simulink model "furuta_block_model"  (R2026b)
settings: Solver=FixedStepDiscrete  StopTime=5  FixedStep=controlPeriod
model workspace (MAT data in the model file):
  controlPeriod = 0.01
  initialState = [0; 0.174532925199; 0; 0]
  integrationStep = 0.002
  lqrGain = [-0.560244322113 -7.30813603654 -0.304541725168 -0.68699829167]
  maxTorque = 0.03
  plantCoefficients = [0.00019818 0.00016078 0.00016134 0.00013805 0.016934 0.0001 1e-05 0]
  scenarioStimulus = [0 0.0075 0.0175 0.0275 0.0375 0.0475 0.0575 0.0675 0.0775 0.0875 0.0975 0.1075 ... (2004 elements, 501x4)]
  usePolicyCallback = 0
values from neighbouring files (symbols this model uses):
  C = [B A*B A^2*B A^3*B]    [build_furuta_rmd.m]
  N = 20    [build_furuta_rl.m]    (also in design_classical.m)
  pidGains = getVariable(mw,'pidGains')    [check_furuta_lqr_capture.m]
  rmd = struct('model','RMD-X6-P20-60-E','voltage',48,'gearRatio',19.612,          'ratedTorque',20,'ratedCurrent',9.5,'ratedSpeedRPM',153,          'noLoadSpeedRPM',176,'Kt',2.1,'currentLSB',.01)    [build_furuta_rmd.m]
  s = load(matFile,'ds')    [analyze_pi_current_run.m]    (also in analyze_pi_speed_run.m; build_furuta_rl.m = sin(x(2));"; build_furuta_simulink.m = s(1); design_classical.m = furuta_scenarios)
  source = [step '/1']    [add_furuta_plant_blocks.m]    (also in build_furuta_pi.m = get_param(line,'SrcPortHandle'); build_furuta_pi_hardware.m = 'Drive interlocks/3'; compare_furuta_actuators.m = get_param([harness '/Requested torque'],'PortHandles'))
  Z = expm([A B; zeros(1,5)]*p.Ts)    [furuta_linearize.m]
undefined symbols (not defined in the file or in its folder): driveElectrical, lmpcF, lmpcH, poleGain, rlRewardLevel, rmdCommandDelaySamples, sgn, useRmd, X, Y
libraries: sm_lib x36, nesl_utility x8, fl_lib x7, rllib x2, mpclib x1, slpidlib x1, ee_lib x1
(part 3 of 4)

== system furuta_block_model/05 Furuta plant/RK4 Furuta plant ==
  state : Inport
  total torque : Inport  Port=2
  Substep 1 : Subsystem
  Substep 2 : Subsystem
  Substep 3 : Subsystem
  Substep 4 : Subsystem
  Substep 5 : Subsystem
  next state : Outport
  wires:
  state/1 -> Substep 1/1(x)
  total torque/1 -> Substep 4/2(tau), Substep 5/2(tau), Substep 3/2(tau), Substep 2/2(tau), Substep 1/2(tau)
  Substep 1/1(x next) -> Substep 2/1(x)
  Substep 2/1(x next) -> Substep 3/1(x)
  Substep 3/1(x next) -> Substep 4/1(x)
  Substep 4/1(x next) -> Substep 5/1(x)
  Substep 5/1(x next) -> next state/1

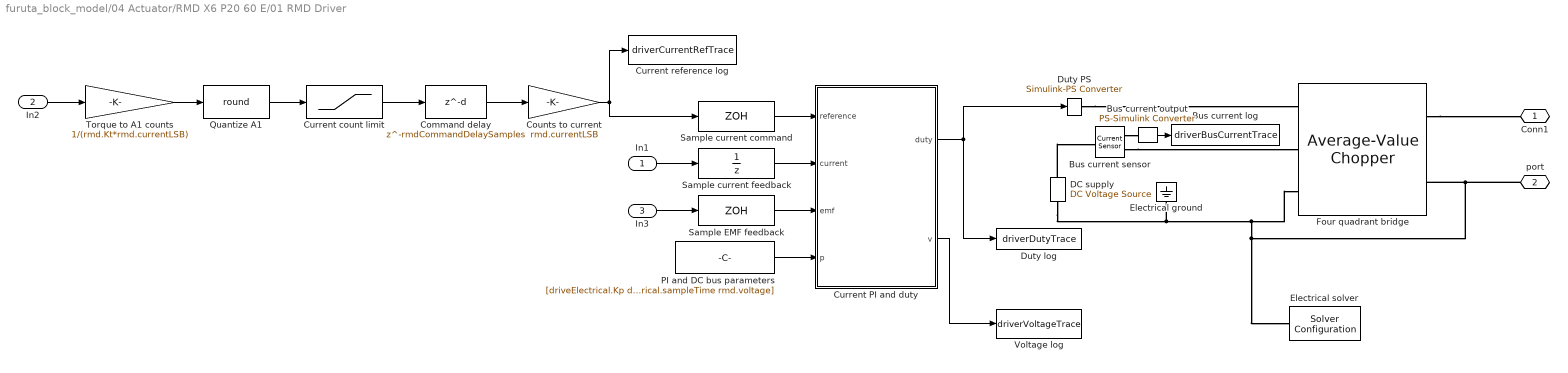
== system furuta_block_model/04 Actuator/RMD X6 P20 60 E/01 RMD Driver ==
  In1 : Inport
  In2 : Inport  Port=2
  In3 : Inport  Port=3
  Bus current log : ToWorkspace  VariableName=driverBusCurrentTrace  SaveFormat=Timeseries  SampleTime=-1
  Bus current output : nesl_utility/PS-Simulink Converter  PhysicalDomain=network_engine_domain  SubClassName=ps_output  LeftPortType=input  RightPortType=output  PseudoPeriodic=off  Frequencies=[]  VectorFormat=inherit  Unit=A  AffineConversion=off
  Bus current sensor : fl_lib/Electrical/Electrical Sensors/Current Sensor
  Command delay : Delay  DelayLength=rmdCommandDelaySamples  SampleTime=controlPeriod
  Counts to current : Gain  Gain=rmd.currentLSB
  Current PI and duty : MATLAB Function  TreatAsAtomicUnit=on
  Current count limit : Saturate  UpperLimit=floor(min([maxTorque/rmd.Kt rmd.ratedTorque/rmd.Kt rmd.ratedCurrent])/rmd.currentLSB)  LowerLimit=-(floor(min([maxTorque/rmd.Kt rmd.ratedTorque/rmd.Kt rmd.ratedCurrent])/rmd.currentLSB))
  Current reference log : ToWorkspace  VariableName=driverCurrentRefTrace  SaveFormat=Timeseries  SampleTime=-1
  DC supply : fl_lib/Electrical/Electrical Sources/DC Voltage Source  v0=rmd.voltage V
  Duty PS : nesl_utility/Simulink-PS Converter  PhysicalDomain=network_engine_domain  SubClassName=ps_input  LeftPortType=input  RightPortType=output  PseudoPeriodic=off  Frequencies=[]  NoiseDistribution=none  NoiseParameters=[]  Unit=1  AffineConversion=off  FilteringAndDerivatives=zero  SimscapeFilterOrder=1  InputFilterTimeConstant=0.001  UdotUserProvided=0
  Duty log : ToWorkspace  VariableName=driverDutyTrace  SaveFormat=Timeseries  SampleTime=-1
  Electrical ground : fl_lib/Electrical/Electrical Elements/Electrical Reference
  Electrical solver : nesl_utility/Solver Configuration  PhysicalDomain=network_engine_domain  SubClassName=solver  LeftPortType=input  RightPortType=generic  Tones=[]  Harmonics=[]  SimulateNoise=off  Profile=off  UseLocalSampling=off  EnableSwitchedLinearOptims=on  FrequencyDomain=off  UseCCode=off  RelTol=0.001  AbsTol=0.001  MinStep=1e-09  ToWorkspace=off  RevertToSquareIcSolve=off  NumHomotopyIterations=100  PhasorMode=off  PhasorModeNumHarmonics=1  ConsistencySolver=NEWTON_XTOL_AFTER_FTOL  CanonicalOrdering=CANONICAL  OptimizeIntermediates=OPTIMIZED  MulticoreSolverChoice=BACKWARD_EULER  IndexReductionMethod=DerivativeReplacement  DoDC=off  ResidualTolerance=1e-09  ConsistencyTolSource=GLOBAL  ConsistencyAbsTol=0.001  ConsistencyRelTol=0.001  ConsistencyTolFactor=0.001  UseLocalSolver=off  LocalSolverChoice=NE_BACKWARD_EULER_ADVANCER  ResolveIndetEquations=on  FunctionEvalNumThread=1  LocalSolverSampleTime=0.001  DoFixedCost=off  MaxNonlinIter=3  MaxModeIter=2  ComputeImpulses=off  ImpulseIterations=2  LinearAlgebra=auto  LinearAlgebraNumThread=0  EquationFormulation=NE_TIME_EF  DelaysMemoryBudget=1024  AutomaticFiltering=on  FilteringTimeConstant=0.001  PartitionStorageMethod=AS_NEEDED  PartitionMemoryBudget=1024  PartitionMethod=BALANCED  MultibodyUseLocalSolver=off  MultibodyLocalSolverChoice=ODE1  MultibodyLocalSolverSampleTime=0.001
  Four quadrant bridge : ee_lib/Semiconductors & Converters/Converters/Average-Value Chopper  chopper_type=ee.enum.converters.averageChopperType.classE  efficiency_option=ee.enum.converters.efficiencyOption.constant  efficiency_fixed=100  i_vec=[0, 2, 5] A  efficiency_vec=[90, 95, 98]
  PI and DC bus parameters : Constant  Value=[driveElectrical.Kp driveElectrical.Ki driveElectrical.sampleTime rmd.voltage]
  Quantize A1 : Rounding  Operator=round
  Sample EMF feedback : ZeroOrderHold  SampleTime=driveElectrical.sampleTime
  Sample current command : ZeroOrderHold  SampleTime=driveElectrical.sampleTime
  Sample current feedback : UnitDelay  SampleTime=driveElectrical.sampleTime
  Torque to A1 counts : Gain  Gain=1/(rmd.Kt*rmd.currentLSB)
  Voltage log : ToWorkspace  VariableName=driverVoltageTrace  SaveFormat=Timeseries  SampleTime=-1
  Conn1 : PMIOPort  Side=Right
  port : PMIOPort  Port=2  Side=Left
  wires:
  Torque to A1 counts/1 -> Quantize A1/1
  Command delay/1 -> Counts to current/1
  Bus current output/1 -> Bus current log/1
  Sample current command/1 -> Current PI and duty/1(reference)
  Counts to current/1 -> Current reference log/1, Sample current command/1
  Current count limit/1 -> Command delay/1
  Quantize A1/1 -> Current count limit/1
  Current PI and duty/1(duty) -> Duty PS/1, Duty log/1
  Sample current feedback/1 -> Current PI and duty/2(current)
  In3/1 -> Sample EMF feedback/1
  Current PI and duty/2(v) -> Voltage log/1
  Sample EMF feedback/1 -> Current PI and duty/3(emf)
  PI and DC bus parameters/1 -> Current PI and duty/4(p)
  In1/1 -> Sample current feedback/1
  In2/1 -> Torque to A1 counts/1
  connections:
  Bus current sensor/RConn1 -- Bus current output/LConn1
  port/RConn1 -- Four quadrant bridge/RConn2 -- Electrical solver/RConn1 -- Four quadrant bridge/LConn3 -- DC supply/RConn1 -- Electrical ground/LConn1
  Duty PS/RConn1 -- Four quadrant bridge/LConn1
  DC supply/LConn1 -- Bus current sensor/LConn1
  Bus current sensor/RConn2 -- Four quadrant bridge/LConn2
  Four quadrant bridge/RConn1 -- Conn1/RConn1

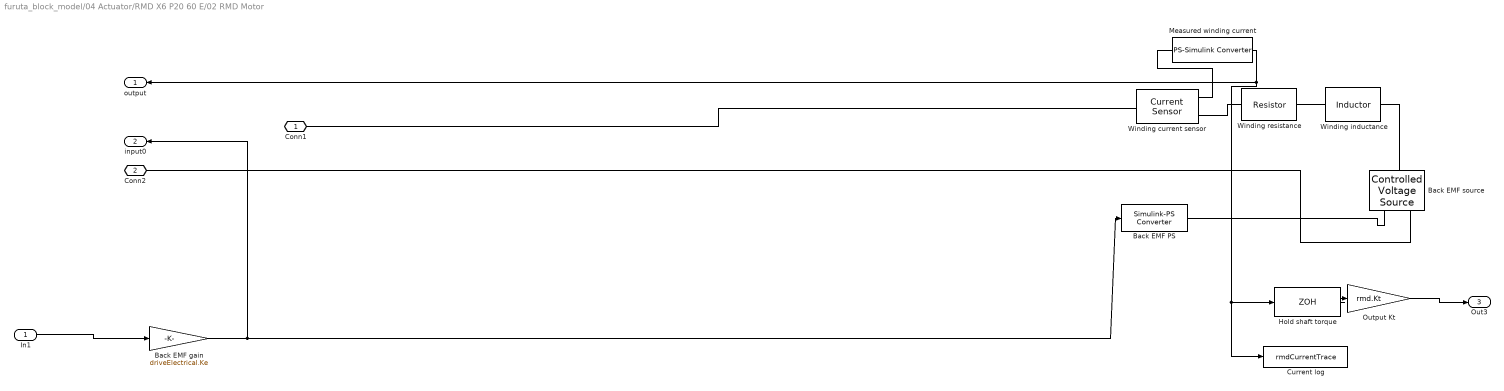
== system furuta_block_model/04 Actuator/RMD X6 P20 60 E/02 RMD Motor ==
  In1 : Inport
  Back EMF PS : nesl_utility/Simulink-PS Converter  PhysicalDomain=network_engine_domain  SubClassName=ps_input  LeftPortType=input  RightPortType=output  PseudoPeriodic=off  Frequencies=[]  NoiseDistribution=none  NoiseParameters=[]  Unit=V  AffineConversion=off  FilteringAndDerivatives=zero  SimscapeFilterOrder=1  InputFilterTimeConstant=0.001  UdotUserProvided=0
  Back EMF gain : Gain  Gain=driveElectrical.Ke
  Back EMF source : fl_lib/Electrical/Electrical Sources/Controlled Voltage Source
  Current log : ToWorkspace  VariableName=rmdCurrentTrace  SampleTime=-1
  Hold shaft torque : ZeroOrderHold  SampleTime=controlPeriod
  Measured winding current : nesl_utility/PS-Simulink Converter  PhysicalDomain=network_engine_domain  SubClassName=ps_output  LeftPortType=input  RightPortType=output  PseudoPeriodic=off  Frequencies=[]  VectorFormat=inherit  Unit=A  AffineConversion=off
  Output Kt : Gain  Gain=rmd.Kt
  Winding current sensor : fl_lib/Electrical/Electrical Sensors/Current Sensor
  Winding inductance : fl_lib/Electrical/Electrical Elements/Inductor  l=driveElectrical.L H  r=0 Ohm  g=0 1/Ohm  i_specify=off  i_priority=None  i=0 A  i_nominal_specify=off  i_nominal_value=1  i_nominal_unit=A  v_specify=off  v_priority=None  v=0 V  v_nominal_specify=off  v_nominal_value=1  v_nominal_unit=V  i_L_specify=off  i_L_priority=High  i_L=0 A  i_L_nominal_specify=off  i_L_nominal_value=1  i_L_nominal_unit=A
  Winding resistance : fl_lib/Electrical/Electrical Elements/Resistor  R=driveElectrical.R Ohm  i_specify=off  i_priority=None  i=0 A  i_nominal_specify=off  i_nominal_value=1  i_nominal_unit=A  v_specify=off  v_priority=None  v=0 V  v_nominal_specify=off  v_nominal_value=1  v_nominal_unit=V
  Conn1 : PMIOPort  Side=Left
  Conn2 : PMIOPort  Port=2  Side=Right
  output : Outport
  input0 : Outport  Port=2
  Out3 : Outport  Port=3
  wires:
  Measured winding current/1 -> output/1, Hold shaft torque/1, Current log/1
  Output Kt/1 -> Out3/1
  Hold shaft torque/1 -> Output Kt/1
  Back EMF gain/1 -> Back EMF PS/1, input0/1
  In1/1 -> Back EMF gain/1
  connections:
  Back EMF PS/RConn1 -- Back EMF source/RConn1
  Winding current sensor/RConn1 -- Measured winding current/LConn1
  Winding resistance/RConn1 -- Winding inductance/LConn1
  Winding inductance/RConn1 -- Back EMF source/LConn1
  Winding current sensor/RConn2 -- Winding resistance/LConn1
  Conn1/RConn1 -- Winding current sensor/LConn1
  Back EMF source/RConn2 -- Conn2/RConn1

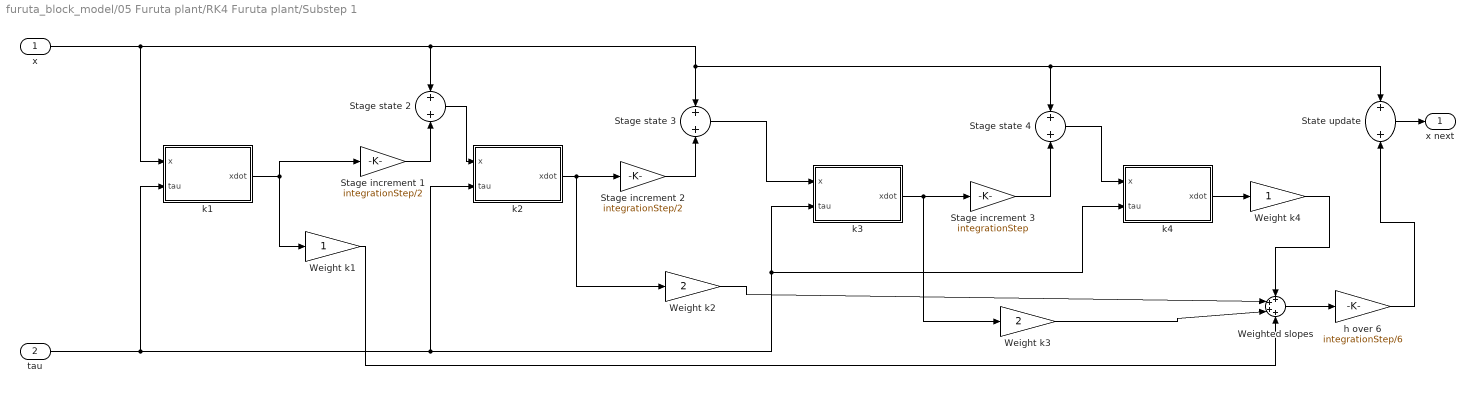
== system furuta_block_model/05 Furuta plant/RK4 Furuta plant/Substep 1 ==
  x : Inport
  tau : Inport  Port=2
  Stage increment 1 : Gain  Gain=integrationStep/2
  Stage increment 2 : Gain  Gain=integrationStep/2
  Stage increment 3 : Gain  Gain=integrationStep
  Stage state 2 : Sum
  Stage state 3 : Sum
  Stage state 4 : Sum
  State update : Sum
  Weight k1 : Gain
  Weight k2 : Gain  Gain=2
  Weight k3 : Gain  Gain=2
  Weight k4 : Gain
  Weighted slopes : Sum  Inputs=++++
  h over 6 : Gain  Gain=integrationStep/6
  k1 : Subsystem
  k2 : Subsystem
  k3 : Subsystem
  k4 : Subsystem
  x next : Outport
  wires:
  x/1 -> Stage state 3/1, Stage state 4/1, State update/1, Stage state 2/1, k1/1(x)
  tau/1 -> k4/2(tau), k3/2(tau), k2/2(tau), k1/2(tau)
  k1/1(xdot) -> Stage increment 1/1, Weight k1/1
  Stage increment 1/1 -> Stage state 2/2
  Stage state 2/1 -> k2/1(x)
  k2/1(xdot) -> Stage increment 2/1, Weight k2/1
  Stage increment 2/1 -> Stage state 3/2
  Stage state 3/1 -> k3/1(x)
  k3/1(xdot) -> Weight k3/1, Stage increment 3/1
  Stage increment 3/1 -> Stage state 4/2
  Stage state 4/1 -> k4/1(x)
  k4/1(xdot) -> Weight k4/1
  Weight k1/1 -> Weighted slopes/4
  Weight k2/1 -> Weighted slopes/2
  Weight k3/1 -> Weighted slopes/3
  Weight k4/1 -> Weighted slopes/1
  Weighted slopes/1 -> h over 6/1
  h over 6/1 -> State update/2
  State update/1 -> x next/1

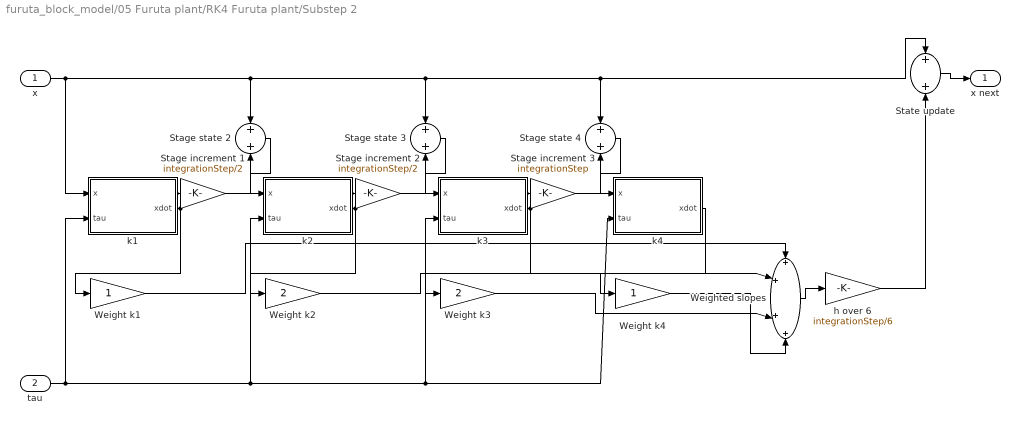
== system furuta_block_model/05 Furuta plant/RK4 Furuta plant/Substep 2 ==
  x : Inport
  tau : Inport  Port=2
  Stage increment 1 : Gain  Gain=integrationStep/2
  Stage increment 2 : Gain  Gain=integrationStep/2
  Stage increment 3 : Gain  Gain=integrationStep
  Stage state 2 : Sum
  Stage state 3 : Sum
  Stage state 4 : Sum
  State update : Sum
  Weight k1 : Gain
  Weight k2 : Gain  Gain=2
  Weight k3 : Gain  Gain=2
  Weight k4 : Gain
  Weighted slopes : Sum  Inputs=++++
  h over 6 : Gain  Gain=integrationStep/6
  k1 : Subsystem
  k2 : Subsystem
  k3 : Subsystem
  k4 : Subsystem
  x next : Outport
  wires:
  State update/1 -> x next/1
  h over 6/1 -> State update/2
  Weighted slopes/1 -> h over 6/1
  Weight k4/1 -> Weighted slopes/4
  Weight k3/1 -> Weighted slopes/3
  Weight k2/1 -> Weighted slopes/2
  Weight k1/1 -> Weighted slopes/1
  k4/1(xdot) -> Weight k4/1
  Stage state 4/1 -> k4/1(x)
  Stage increment 3/1 -> Stage state 4/2
  k3/1(xdot) -> Weight k3/1, Stage increment 3/1
  Stage state 3/1 -> k3/1(x)
  Stage increment 2/1 -> Stage state 3/2
  k2/1(xdot) -> Weight k2/1, Stage increment 2/1
  Stage state 2/1 -> k2/1(x)
  Stage increment 1/1 -> Stage state 2/2
  k1/1(xdot) -> Weight k1/1, Stage increment 1/1
  tau/1 -> k4/2(tau), k3/2(tau), k2/2(tau), k1/2(tau)
  x/1 -> State update/1, Stage state 4/1, Stage state 3/1, Stage state 2/1, k1/1(x)

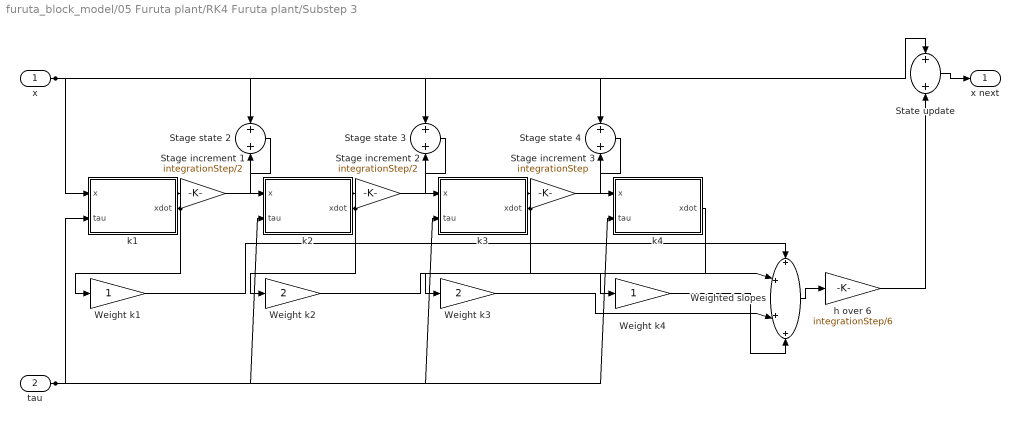
== system furuta_block_model/05 Furuta plant/RK4 Furuta plant/Substep 3 ==
  x : Inport
  tau : Inport  Port=2
  Stage increment 1 : Gain  Gain=integrationStep/2
  Stage increment 2 : Gain  Gain=integrationStep/2
  Stage increment 3 : Gain  Gain=integrationStep
  Stage state 2 : Sum
  Stage state 3 : Sum
  Stage state 4 : Sum
  State update : Sum
  Weight k1 : Gain
  Weight k2 : Gain  Gain=2
  Weight k3 : Gain  Gain=2
  Weight k4 : Gain
  Weighted slopes : Sum  Inputs=++++
  h over 6 : Gain  Gain=integrationStep/6
  k1 : Subsystem
  k2 : Subsystem
  k3 : Subsystem
  k4 : Subsystem
  x next : Outport
  wires:
  State update/1 -> x next/1
  h over 6/1 -> State update/2
  Weighted slopes/1 -> h over 6/1
  Weight k4/1 -> Weighted slopes/4
  Weight k3/1 -> Weighted slopes/3
  Weight k2/1 -> Weighted slopes/2
  Weight k1/1 -> Weighted slopes/1
  k4/1(xdot) -> Weight k4/1
  Stage state 4/1 -> k4/1(x)
  Stage increment 3/1 -> Stage state 4/2
  k3/1(xdot) -> Weight k3/1, Stage increment 3/1
  Stage state 3/1 -> k3/1(x)
  Stage increment 2/1 -> Stage state 3/2
  k2/1(xdot) -> Weight k2/1, Stage increment 2/1
  Stage state 2/1 -> k2/1(x)
  Stage increment 1/1 -> Stage state 2/2
  k1/1(xdot) -> Weight k1/1, Stage increment 1/1
  tau/1 -> k4/2(tau), k3/2(tau), k2/2(tau), k1/2(tau)
  x/1 -> State update/1, Stage state 4/1, Stage state 3/1, Stage state 2/1, k1/1(x)

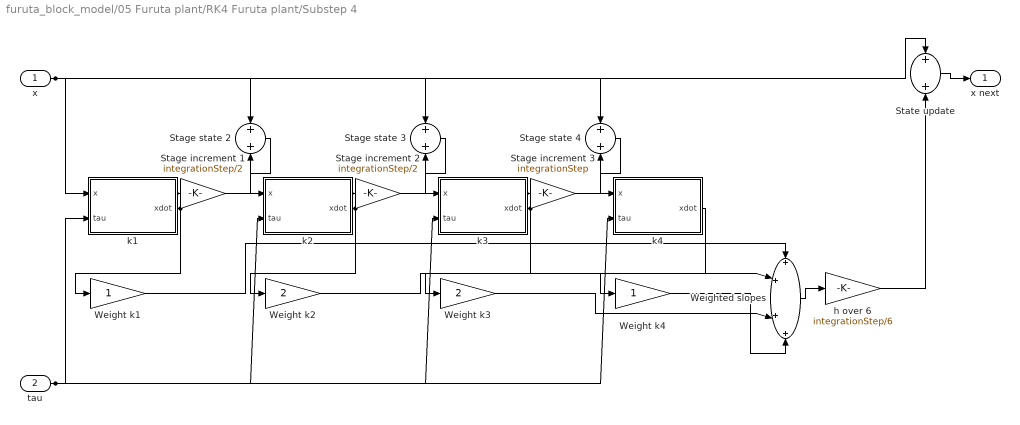
== system furuta_block_model/05 Furuta plant/RK4 Furuta plant/Substep 4 ==
  x : Inport
  tau : Inport  Port=2
  Stage increment 1 : Gain  Gain=integrationStep/2
  Stage increment 2 : Gain  Gain=integrationStep/2
  Stage increment 3 : Gain  Gain=integrationStep
  Stage state 2 : Sum
  Stage state 3 : Sum
  Stage state 4 : Sum
  State update : Sum
  Weight k1 : Gain
  Weight k2 : Gain  Gain=2
  Weight k3 : Gain  Gain=2
  Weight k4 : Gain
  Weighted slopes : Sum  Inputs=++++
  h over 6 : Gain  Gain=integrationStep/6
  k1 : Subsystem
  k2 : Subsystem
  k3 : Subsystem
  k4 : Subsystem
  x next : Outport
  wires:
  State update/1 -> x next/1
  h over 6/1 -> State update/2
  Weighted slopes/1 -> h over 6/1
  Weight k4/1 -> Weighted slopes/4
  Weight k3/1 -> Weighted slopes/3
  Weight k2/1 -> Weighted slopes/2
  Weight k1/1 -> Weighted slopes/1
  k4/1(xdot) -> Weight k4/1
  Stage state 4/1 -> k4/1(x)
  Stage increment 3/1 -> Stage state 4/2
  k3/1(xdot) -> Weight k3/1, Stage increment 3/1
  Stage state 3/1 -> k3/1(x)
  Stage increment 2/1 -> Stage state 3/2
  k2/1(xdot) -> Weight k2/1, Stage increment 2/1
  Stage state 2/1 -> k2/1(x)
  Stage increment 1/1 -> Stage state 2/2
  k1/1(xdot) -> Weight k1/1, Stage increment 1/1
  tau/1 -> k4/2(tau), k3/2(tau), k2/2(tau), k1/2(tau)
  x/1 -> State update/1, Stage state 4/1, Stage state 3/1, Stage state 2/1, k1/1(x)

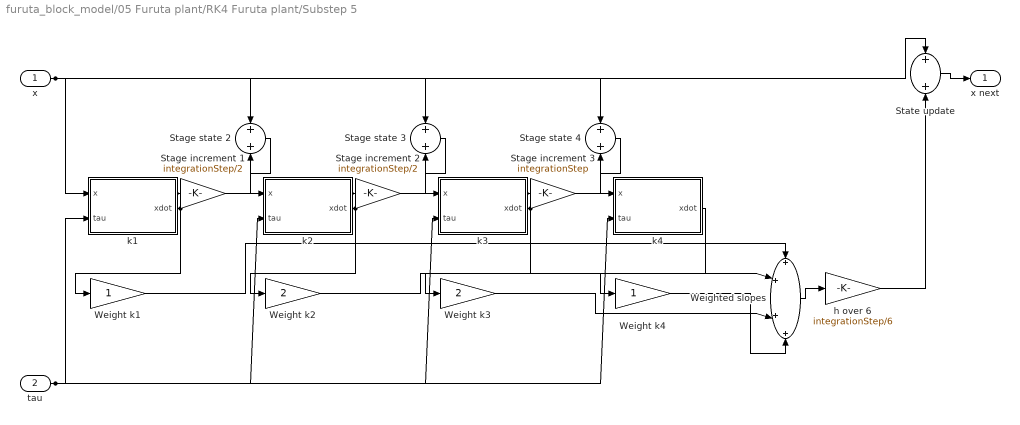
== system furuta_block_model/05 Furuta plant/RK4 Furuta plant/Substep 5 ==
  x : Inport
  tau : Inport  Port=2
  Stage increment 1 : Gain  Gain=integrationStep/2
  Stage increment 2 : Gain  Gain=integrationStep/2
  Stage increment 3 : Gain  Gain=integrationStep
  Stage state 2 : Sum
  Stage state 3 : Sum
  Stage state 4 : Sum
  State update : Sum
  Weight k1 : Gain
  Weight k2 : Gain  Gain=2
  Weight k3 : Gain  Gain=2
  Weight k4 : Gain
  Weighted slopes : Sum  Inputs=++++
  h over 6 : Gain  Gain=integrationStep/6
  k1 : Subsystem
  k2 : Subsystem
  k3 : Subsystem
  k4 : Subsystem
  x next : Outport
  wires:
  State update/1 -> x next/1
  h over 6/1 -> State update/2
  Weighted slopes/1 -> h over 6/1
  Weight k4/1 -> Weighted slopes/4
  Weight k3/1 -> Weighted slopes/3
  Weight k2/1 -> Weighted slopes/2
  Weight k1/1 -> Weighted slopes/1
  k4/1(xdot) -> Weight k4/1
  Stage state 4/1 -> k4/1(x)
  Stage increment 3/1 -> Stage state 4/2
  k3/1(xdot) -> Weight k3/1, Stage increment 3/1
  Stage state 3/1 -> k3/1(x)
  Stage increment 2/1 -> Stage state 3/2
  k2/1(xdot) -> Weight k2/1, Stage increment 2/1
  Stage state 2/1 -> k2/1(x)
  Stage increment 1/1 -> Stage state 2/2
  k1/1(xdot) -> Weight k1/1, Stage increment 1/1
  tau/1 -> k4/2(tau), k3/2(tau), k2/2(tau), k1/2(tau)
  x/1 -> State update/1, Stage state 4/1, Stage state 3/1, Stage state 2/1, k1/1(x)

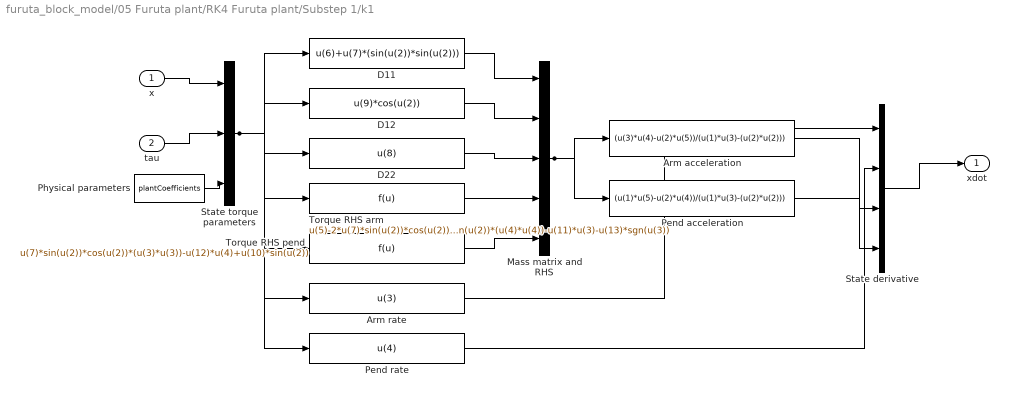
== system furuta_block_model/05 Furuta plant/RK4 Furuta plant/Substep 1/k1 ==
  x : Inport
  tau : Inport  Port=2
  Arm acceleration : Fcn  Expr=(u(3)*u(4)-u(2)*u(5))/(u(1)*u(3)-(u(2)*u(2)))
  Arm rate : Fcn  Expr=u(3)
  D11 : Fcn  Expr=u(6)+u(7)*(sin(u(2))*sin(u(2)))
  D12 : Fcn  Expr=u(9)*cos(u(2))
  D22 : Fcn  Expr=u(8)
  Mass matrix and RHS : Mux  Inputs=5
  Pend acceleration : Fcn  Expr=(u(1)*u(5)-u(2)*u(4))/(u(1)*u(3)-(u(2)*u(2)))
  Pend rate : Fcn  Expr=u(4)
  Physical parameters : Constant  Value=plantCoefficients
  State derivative : Mux
  State torque parameters : Mux  Inputs=3
  Torque RHS arm : Fcn  Expr=u(5)-2*u(7)*sin(u(2))*cos(u(2))*u(3)*u(4)+u(9)*sin(u(2))*(u(4)*u(4))-u(11)*u(3)-u(13)*sgn(u(3))
  Torque RHS pend : Fcn  Expr=u(7)*sin(u(2))*cos(u(2))*(u(3)*u(3))-u(12)*u(4)+u(10)*sin(u(2))
  xdot : Outport
  wires:
  x/1 -> State torque parameters/1
  tau/1 -> State torque parameters/2
  Physical parameters/1 -> State torque parameters/3
  State torque parameters/1 -> D11/1, D12/1, D22/1, Torque RHS arm/1, Torque RHS pend/1, Arm rate/1, Pend rate/1
  D11/1 -> Mass matrix and RHS/1
  D12/1 -> Mass matrix and RHS/2
  D22/1 -> Mass matrix and RHS/3
  Torque RHS arm/1 -> Mass matrix and RHS/4
  Torque RHS pend/1 -> Mass matrix and RHS/5
  Arm rate/1 -> State derivative/1
  Pend rate/1 -> State derivative/2
  Mass matrix and RHS/1 -> Arm acceleration/1, Pend acceleration/1
  Arm acceleration/1 -> State derivative/3
  Pend acceleration/1 -> State derivative/4
  State derivative/1 -> xdot/1

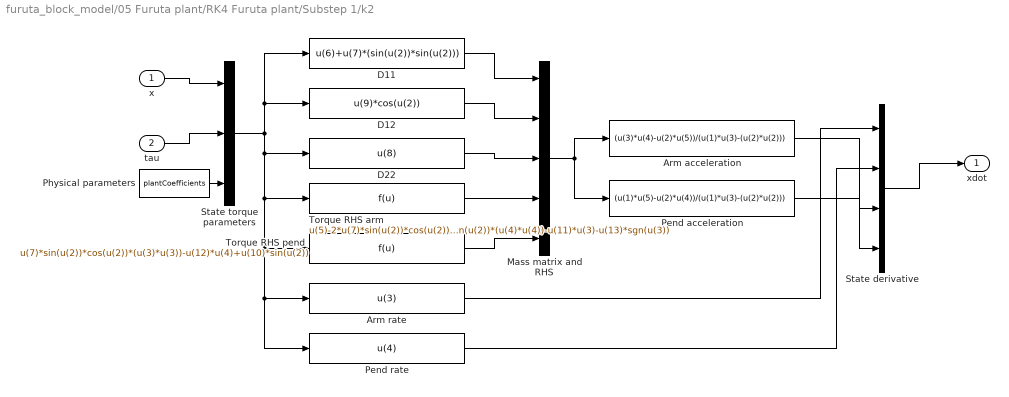
== system furuta_block_model/05 Furuta plant/RK4 Furuta plant/Substep 1/k2 ==
  x : Inport
  tau : Inport  Port=2
  Arm acceleration : Fcn  Expr=(u(3)*u(4)-u(2)*u(5))/(u(1)*u(3)-(u(2)*u(2)))
  Arm rate : Fcn  Expr=u(3)
  D11 : Fcn  Expr=u(6)+u(7)*(sin(u(2))*sin(u(2)))
  D12 : Fcn  Expr=u(9)*cos(u(2))
  D22 : Fcn  Expr=u(8)
  Mass matrix and RHS : Mux  Inputs=5
  Pend acceleration : Fcn  Expr=(u(1)*u(5)-u(2)*u(4))/(u(1)*u(3)-(u(2)*u(2)))
  Pend rate : Fcn  Expr=u(4)
  Physical parameters : Constant  Value=plantCoefficients
  State derivative : Mux
  State torque parameters : Mux  Inputs=3
  Torque RHS arm : Fcn  Expr=u(5)-2*u(7)*sin(u(2))*cos(u(2))*u(3)*u(4)+u(9)*sin(u(2))*(u(4)*u(4))-u(11)*u(3)-u(13)*sgn(u(3))
  Torque RHS pend : Fcn  Expr=u(7)*sin(u(2))*cos(u(2))*(u(3)*u(3))-u(12)*u(4)+u(10)*sin(u(2))
  xdot : Outport
  wires:
  State derivative/1 -> xdot/1
  Pend acceleration/1 -> State derivative/4
  Arm acceleration/1 -> State derivative/3
  Mass matrix and RHS/1 -> Pend acceleration/1, Arm acceleration/1
  Pend rate/1 -> State derivative/2
  Arm rate/1 -> State derivative/1
  Torque RHS pend/1 -> Mass matrix and RHS/5
  Torque RHS arm/1 -> Mass matrix and RHS/4
  D22/1 -> Mass matrix and RHS/3
  D12/1 -> Mass matrix and RHS/2
  D11/1 -> Mass matrix and RHS/1
  State torque parameters/1 -> Pend rate/1, Arm rate/1, Torque RHS pend/1, Torque RHS arm/1, D22/1, D12/1, D11/1
  Physical parameters/1 -> State torque parameters/3
  tau/1 -> State torque parameters/2
  x/1 -> State torque parameters/1

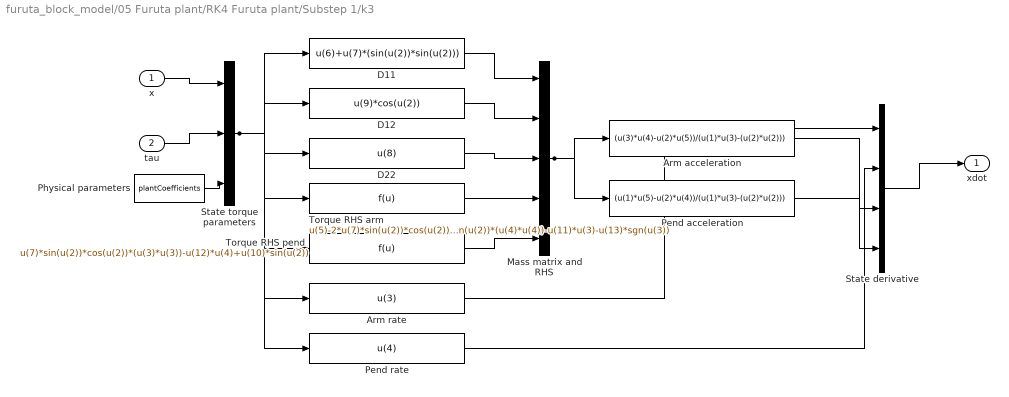
== system furuta_block_model/05 Furuta plant/RK4 Furuta plant/Substep 1/k3 ==
  x : Inport
  tau : Inport  Port=2
  Arm acceleration : Fcn  Expr=(u(3)*u(4)-u(2)*u(5))/(u(1)*u(3)-(u(2)*u(2)))
  Arm rate : Fcn  Expr=u(3)
  D11 : Fcn  Expr=u(6)+u(7)*(sin(u(2))*sin(u(2)))
  D12 : Fcn  Expr=u(9)*cos(u(2))
  D22 : Fcn  Expr=u(8)
  Mass matrix and RHS : Mux  Inputs=5
  Pend acceleration : Fcn  Expr=(u(1)*u(5)-u(2)*u(4))/(u(1)*u(3)-(u(2)*u(2)))
  Pend rate : Fcn  Expr=u(4)
  Physical parameters : Constant  Value=plantCoefficients
  State derivative : Mux
  State torque parameters : Mux  Inputs=3
  Torque RHS arm : Fcn  Expr=u(5)-2*u(7)*sin(u(2))*cos(u(2))*u(3)*u(4)+u(9)*sin(u(2))*(u(4)*u(4))-u(11)*u(3)-u(13)*sgn(u(3))
  Torque RHS pend : Fcn  Expr=u(7)*sin(u(2))*cos(u(2))*(u(3)*u(3))-u(12)*u(4)+u(10)*sin(u(2))
  xdot : Outport
  wires:
  State derivative/1 -> xdot/1
  Pend acceleration/1 -> State derivative/4
  Arm acceleration/1 -> State derivative/3
  Mass matrix and RHS/1 -> Pend acceleration/1, Arm acceleration/1
  Pend rate/1 -> State derivative/2
  Arm rate/1 -> State derivative/1
  Torque RHS pend/1 -> Mass matrix and RHS/5
  Torque RHS arm/1 -> Mass matrix and RHS/4
  D22/1 -> Mass matrix and RHS/3
  D12/1 -> Mass matrix and RHS/2
  D11/1 -> Mass matrix and RHS/1
  State torque parameters/1 -> Pend rate/1, Arm rate/1, Torque RHS pend/1, Torque RHS arm/1, D22/1, D12/1, D11/1
  Physical parameters/1 -> State torque parameters/3
  tau/1 -> State torque parameters/2
  x/1 -> State torque parameters/1

== system furuta_block_model/05 Furuta plant/RK4 Furuta plant/Substep 1/k4 ==
  x : Inport
  tau : Inport  Port=2
  Arm acceleration : Fcn  Expr=(u(3)*u(4)-u(2)*u(5))/(u(1)*u(3)-(u(2)*u(2)))
  Arm rate : Fcn  Expr=u(3)
  D11 : Fcn  Expr=u(6)+u(7)*(sin(u(2))*sin(u(2)))
  D12 : Fcn  Expr=u(9)*cos(u(2))
  D22 : Fcn  Expr=u(8)
  Mass matrix and RHS : Mux  Inputs=5
  Pend acceleration : Fcn  Expr=(u(1)*u(5)-u(2)*u(4))/(u(1)*u(3)-(u(2)*u(2)))
  Pend rate : Fcn  Expr=u(4)
  Physical parameters : Constant  Value=plantCoefficients
  State derivative : Mux
  State torque parameters : Mux  Inputs=3
  Torque RHS arm : Fcn  Expr=u(5)-2*u(7)*sin(u(2))*cos(u(2))*u(3)*u(4)+u(9)*sin(u(2))*(u(4)*u(4))-u(11)*u(3)-u(13)*sgn(u(3))
  Torque RHS pend : Fcn  Expr=u(7)*sin(u(2))*cos(u(2))*(u(3)*u(3))-u(12)*u(4)+u(10)*sin(u(2))
  xdot : Outport
  wires:
  State derivative/1 -> xdot/1
  Pend acceleration/1 -> State derivative/4
  Arm acceleration/1 -> State derivative/3
  Mass matrix and RHS/1 -> Pend acceleration/1, Arm acceleration/1
  Pend rate/1 -> State derivative/2
  Arm rate/1 -> State derivative/1
  Torque RHS pend/1 -> Mass matrix and RHS/5
  Torque RHS arm/1 -> Mass matrix and RHS/4
  D22/1 -> Mass matrix and RHS/3
  D12/1 -> Mass matrix and RHS/2
  D11/1 -> Mass matrix and RHS/1
  State torque parameters/1 -> Pend rate/1, Arm rate/1, Torque RHS pend/1, Torque RHS arm/1, D22/1, D12/1, D11/1
  Physical parameters/1 -> State torque parameters/3
  tau/1 -> State torque parameters/2
  x/1 -> State torque parameters/1

== system furuta_block_model/05 Furuta plant/RK4 Furuta plant/Substep 2/k1 ==
  x : Inport
  tau : Inport  Port=2
  Arm acceleration : Fcn  Expr=(u(3)*u(4)-u(2)*u(5))/(u(1)*u(3)-(u(2)*u(2)))
  Arm rate : Fcn  Expr=u(3)
  D11 : Fcn  Expr=u(6)+u(7)*(sin(u(2))*sin(u(2)))
  D12 : Fcn  Expr=u(9)*cos(u(2))
  D22 : Fcn  Expr=u(8)
  Mass matrix and RHS : Mux  Inputs=5
  Pend acceleration : Fcn  Expr=(u(1)*u(5)-u(2)*u(4))/(u(1)*u(3)-(u(2)*u(2)))
  Pend rate : Fcn  Expr=u(4)
  Physical parameters : Constant  Value=plantCoefficients
  State derivative : Mux
  State torque parameters : Mux  Inputs=3
  Torque RHS arm : Fcn  Expr=u(5)-2*u(7)*sin(u(2))*cos(u(2))*u(3)*u(4)+u(9)*sin(u(2))*(u(4)*u(4))-u(11)*u(3)-u(13)*sgn(u(3))
  Torque RHS pend : Fcn  Expr=u(7)*sin(u(2))*cos(u(2))*(u(3)*u(3))-u(12)*u(4)+u(10)*sin(u(2))
  xdot : Outport
  wires:
  State derivative/1 -> xdot/1
  Pend acceleration/1 -> State derivative/4
  Arm acceleration/1 -> State derivative/3
  Mass matrix and RHS/1 -> Pend acceleration/1, Arm acceleration/1
  Pend rate/1 -> State derivative/2
  Arm rate/1 -> State derivative/1
  Torque RHS pend/1 -> Mass matrix and RHS/5
  Torque RHS arm/1 -> Mass matrix and RHS/4
  D22/1 -> Mass matrix and RHS/3
  D12/1 -> Mass matrix and RHS/2
  D11/1 -> Mass matrix and RHS/1
  State torque parameters/1 -> Pend rate/1, Arm rate/1, Torque RHS pend/1, Torque RHS arm/1, D22/1, D12/1, D11/1
  Physical parameters/1 -> State torque parameters/3
  tau/1 -> State torque parameters/2
  x/1 -> State torque parameters/1

== system furuta_block_model/05 Furuta plant/RK4 Furuta plant/Substep 2/k2 ==
  x : Inport
  tau : Inport  Port=2
  Arm acceleration : Fcn  Expr=(u(3)*u(4)-u(2)*u(5))/(u(1)*u(3)-(u(2)*u(2)))
  Arm rate : Fcn  Expr=u(3)
  D11 : Fcn  Expr=u(6)+u(7)*(sin(u(2))*sin(u(2)))
  D12 : Fcn  Expr=u(9)*cos(u(2))
  D22 : Fcn  Expr=u(8)
  Mass matrix and RHS : Mux  Inputs=5
  Pend acceleration : Fcn  Expr=(u(1)*u(5)-u(2)*u(4))/(u(1)*u(3)-(u(2)*u(2)))
  Pend rate : Fcn  Expr=u(4)
  Physical parameters : Constant  Value=plantCoefficients
  State derivative : Mux
  State torque parameters : Mux  Inputs=3
  Torque RHS arm : Fcn  Expr=u(5)-2*u(7)*sin(u(2))*cos(u(2))*u(3)*u(4)+u(9)*sin(u(2))*(u(4)*u(4))-u(11)*u(3)-u(13)*sgn(u(3))
  Torque RHS pend : Fcn  Expr=u(7)*sin(u(2))*cos(u(2))*(u(3)*u(3))-u(12)*u(4)+u(10)*sin(u(2))
  xdot : Outport
  wires:
  x/1 -> State torque parameters/1
  tau/1 -> State torque parameters/2
  Physical parameters/1 -> State torque parameters/3
  State torque parameters/1 -> D11/1, D12/1, D22/1, Torque RHS arm/1, Torque RHS pend/1, Arm rate/1, Pend rate/1
  D11/1 -> Mass matrix and RHS/1
  D12/1 -> Mass matrix and RHS/2
  D22/1 -> Mass matrix and RHS/3
  Torque RHS arm/1 -> Mass matrix and RHS/4
  Torque RHS pend/1 -> Mass matrix and RHS/5
  Arm rate/1 -> State derivative/1
  Pend rate/1 -> State derivative/2
  Mass matrix and RHS/1 -> Arm acceleration/1, Pend acceleration/1
  Arm acceleration/1 -> State derivative/3
  Pend acceleration/1 -> State derivative/4
  State derivative/1 -> xdot/1

== system furuta_block_model/05 Furuta plant/RK4 Furuta plant/Substep 2/k3 ==
  x : Inport
  tau : Inport  Port=2
  Arm acceleration : Fcn  Expr=(u(3)*u(4)-u(2)*u(5))/(u(1)*u(3)-(u(2)*u(2)))
  Arm rate : Fcn  Expr=u(3)
  D11 : Fcn  Expr=u(6)+u(7)*(sin(u(2))*sin(u(2)))
  D12 : Fcn  Expr=u(9)*cos(u(2))
  D22 : Fcn  Expr=u(8)
  Mass matrix and RHS : Mux  Inputs=5
  Pend acceleration : Fcn  Expr=(u(1)*u(5)-u(2)*u(4))/(u(1)*u(3)-(u(2)*u(2)))
  Pend rate : Fcn  Expr=u(4)
  Physical parameters : Constant  Value=plantCoefficients
  State derivative : Mux
  State torque parameters : Mux  Inputs=3
  Torque RHS arm : Fcn  Expr=u(5)-2*u(7)*sin(u(2))*cos(u(2))*u(3)*u(4)+u(9)*sin(u(2))*(u(4)*u(4))-u(11)*u(3)-u(13)*sgn(u(3))
  Torque RHS pend : Fcn  Expr=u(7)*sin(u(2))*cos(u(2))*(u(3)*u(3))-u(12)*u(4)+u(10)*sin(u(2))
  xdot : Outport
  wires:
  x/1 -> State torque parameters/1
  tau/1 -> State torque parameters/2
  Physical parameters/1 -> State torque parameters/3
  State torque parameters/1 -> D11/1, D12/1, D22/1, Torque RHS arm/1, Torque RHS pend/1, Arm rate/1, Pend rate/1
  D11/1 -> Mass matrix and RHS/1
  D12/1 -> Mass matrix and RHS/2
  D22/1 -> Mass matrix and RHS/3
  Torque RHS arm/1 -> Mass matrix and RHS/4
  Torque RHS pend/1 -> Mass matrix and RHS/5
  Arm rate/1 -> State derivative/1
  Pend rate/1 -> State derivative/2
  Mass matrix and RHS/1 -> Arm acceleration/1, Pend acceleration/1
  Arm acceleration/1 -> State derivative/3
  Pend acceleration/1 -> State derivative/4
  State derivative/1 -> xdot/1

== system furuta_block_model/05 Furuta plant/RK4 Furuta plant/Substep 2/k4 ==
  x : Inport
  tau : Inport  Port=2
  Arm acceleration : Fcn  Expr=(u(3)*u(4)-u(2)*u(5))/(u(1)*u(3)-(u(2)*u(2)))
  Arm rate : Fcn  Expr=u(3)
  D11 : Fcn  Expr=u(6)+u(7)*(sin(u(2))*sin(u(2)))
  D12 : Fcn  Expr=u(9)*cos(u(2))
  D22 : Fcn  Expr=u(8)
  Mass matrix and RHS : Mux  Inputs=5
  Pend acceleration : Fcn  Expr=(u(1)*u(5)-u(2)*u(4))/(u(1)*u(3)-(u(2)*u(2)))
  Pend rate : Fcn  Expr=u(4)
  Physical parameters : Constant  Value=plantCoefficients
  State derivative : Mux
  State torque parameters : Mux  Inputs=3
  Torque RHS arm : Fcn  Expr=u(5)-2*u(7)*sin(u(2))*cos(u(2))*u(3)*u(4)+u(9)*sin(u(2))*(u(4)*u(4))-u(11)*u(3)-u(13)*sgn(u(3))
  Torque RHS pend : Fcn  Expr=u(7)*sin(u(2))*cos(u(2))*(u(3)*u(3))-u(12)*u(4)+u(10)*sin(u(2))
  xdot : Outport
  wires:
  x/1 -> State torque parameters/1
  tau/1 -> State torque parameters/2
  Physical parameters/1 -> State torque parameters/3
  State torque parameters/1 -> D11/1, D12/1, D22/1, Torque RHS arm/1, Torque RHS pend/1, Arm rate/1, Pend rate/1
  D11/1 -> Mass matrix and RHS/1
  D12/1 -> Mass matrix and RHS/2
  D22/1 -> Mass matrix and RHS/3
  Torque RHS arm/1 -> Mass matrix and RHS/4
  Torque RHS pend/1 -> Mass matrix and RHS/5
  Arm rate/1 -> State derivative/1
  Pend rate/1 -> State derivative/2
  Mass matrix and RHS/1 -> Arm acceleration/1, Pend acceleration/1
  Arm acceleration/1 -> State derivative/3
  Pend acceleration/1 -> State derivative/4
  State derivative/1 -> xdot/1

== system furuta_block_model/05 Furuta plant/RK4 Furuta plant/Substep 3/k1 ==
  x : Inport
  tau : Inport  Port=2
  Arm acceleration : Fcn  Expr=(u(3)*u(4)-u(2)*u(5))/(u(1)*u(3)-(u(2)*u(2)))
  Arm rate : Fcn  Expr=u(3)
  D11 : Fcn  Expr=u(6)+u(7)*(sin(u(2))*sin(u(2)))
  D12 : Fcn  Expr=u(9)*cos(u(2))
  D22 : Fcn  Expr=u(8)
  Mass matrix and RHS : Mux  Inputs=5
  Pend acceleration : Fcn  Expr=(u(1)*u(5)-u(2)*u(4))/(u(1)*u(3)-(u(2)*u(2)))
  Pend rate : Fcn  Expr=u(4)
  Physical parameters : Constant  Value=plantCoefficients
  State derivative : Mux
  State torque parameters : Mux  Inputs=3
  Torque RHS arm : Fcn  Expr=u(5)-2*u(7)*sin(u(2))*cos(u(2))*u(3)*u(4)+u(9)*sin(u(2))*(u(4)*u(4))-u(11)*u(3)-u(13)*sgn(u(3))
  Torque RHS pend : Fcn  Expr=u(7)*sin(u(2))*cos(u(2))*(u(3)*u(3))-u(12)*u(4)+u(10)*sin(u(2))
  xdot : Outport
  wires:
  State derivative/1 -> xdot/1
  Pend acceleration/1 -> State derivative/4
  Arm acceleration/1 -> State derivative/3
  Mass matrix and RHS/1 -> Pend acceleration/1, Arm acceleration/1
  Pend rate/1 -> State derivative/2
  Arm rate/1 -> State derivative/1
  Torque RHS pend/1 -> Mass matrix and RHS/5
  Torque RHS arm/1 -> Mass matrix and RHS/4
  D22/1 -> Mass matrix and RHS/3
  D12/1 -> Mass matrix and RHS/2
  D11/1 -> Mass matrix and RHS/1
  State torque parameters/1 -> Pend rate/1, Arm rate/1, Torque RHS pend/1, Torque RHS arm/1, D22/1, D12/1, D11/1
  Physical parameters/1 -> State torque parameters/3
  tau/1 -> State torque parameters/2
  x/1 -> State torque parameters/1

== system furuta_block_model/05 Furuta plant/RK4 Furuta plant/Substep 3/k2 ==
  x : Inport
  tau : Inport  Port=2
  Arm acceleration : Fcn  Expr=(u(3)*u(4)-u(2)*u(5))/(u(1)*u(3)-(u(2)*u(2)))
  Arm rate : Fcn  Expr=u(3)
  D11 : Fcn  Expr=u(6)+u(7)*(sin(u(2))*sin(u(2)))
  D12 : Fcn  Expr=u(9)*cos(u(2))
  D22 : Fcn  Expr=u(8)
  Mass matrix and RHS : Mux  Inputs=5
  Pend acceleration : Fcn  Expr=(u(1)*u(5)-u(2)*u(4))/(u(1)*u(3)-(u(2)*u(2)))
  Pend rate : Fcn  Expr=u(4)
  Physical parameters : Constant  Value=plantCoefficients
  State derivative : Mux
  State torque parameters : Mux  Inputs=3
  Torque RHS arm : Fcn  Expr=u(5)-2*u(7)*sin(u(2))*cos(u(2))*u(3)*u(4)+u(9)*sin(u(2))*(u(4)*u(4))-u(11)*u(3)-u(13)*sgn(u(3))
  Torque RHS pend : Fcn  Expr=u(7)*sin(u(2))*cos(u(2))*(u(3)*u(3))-u(12)*u(4)+u(10)*sin(u(2))
  xdot : Outport
  wires:
  x/1 -> State torque parameters/1
  tau/1 -> State torque parameters/2
  Physical parameters/1 -> State torque parameters/3
  State torque parameters/1 -> D11/1, D12/1, D22/1, Torque RHS arm/1, Torque RHS pend/1, Arm rate/1, Pend rate/1
  D11/1 -> Mass matrix and RHS/1
  D12/1 -> Mass matrix and RHS/2
  D22/1 -> Mass matrix and RHS/3
  Torque RHS arm/1 -> Mass matrix and RHS/4
  Torque RHS pend/1 -> Mass matrix and RHS/5
  Arm rate/1 -> State derivative/1
  Pend rate/1 -> State derivative/2
  Mass matrix and RHS/1 -> Arm acceleration/1, Pend acceleration/1
  Arm acceleration/1 -> State derivative/3
  Pend acceleration/1 -> State derivative/4
  State derivative/1 -> xdot/1

== system furuta_block_model/05 Furuta plant/RK4 Furuta plant/Substep 3/k3 ==
  x : Inport
  tau : Inport  Port=2
  Arm acceleration : Fcn  Expr=(u(3)*u(4)-u(2)*u(5))/(u(1)*u(3)-(u(2)*u(2)))
  Arm rate : Fcn  Expr=u(3)
  D11 : Fcn  Expr=u(6)+u(7)*(sin(u(2))*sin(u(2)))
  D12 : Fcn  Expr=u(9)*cos(u(2))
  D22 : Fcn  Expr=u(8)
  Mass matrix and RHS : Mux  Inputs=5
  Pend acceleration : Fcn  Expr=(u(1)*u(5)-u(2)*u(4))/(u(1)*u(3)-(u(2)*u(2)))
  Pend rate : Fcn  Expr=u(4)
  Physical parameters : Constant  Value=plantCoefficients
  State derivative : Mux
  State torque parameters : Mux  Inputs=3
  Torque RHS arm : Fcn  Expr=u(5)-2*u(7)*sin(u(2))*cos(u(2))*u(3)*u(4)+u(9)*sin(u(2))*(u(4)*u(4))-u(11)*u(3)-u(13)*sgn(u(3))
  Torque RHS pend : Fcn  Expr=u(7)*sin(u(2))*cos(u(2))*(u(3)*u(3))-u(12)*u(4)+u(10)*sin(u(2))
  xdot : Outport
  wires:
  x/1 -> State torque parameters/1
  tau/1 -> State torque parameters/2
  Physical parameters/1 -> State torque parameters/3
  State torque parameters/1 -> D11/1, D12/1, D22/1, Torque RHS arm/1, Torque RHS pend/1, Arm rate/1, Pend rate/1
  D11/1 -> Mass matrix and RHS/1
  D12/1 -> Mass matrix and RHS/2
  D22/1 -> Mass matrix and RHS/3
  Torque RHS arm/1 -> Mass matrix and RHS/4
  Torque RHS pend/1 -> Mass matrix and RHS/5
  Arm rate/1 -> State derivative/1
  Pend rate/1 -> State derivative/2
  Mass matrix and RHS/1 -> Arm acceleration/1, Pend acceleration/1
  Arm acceleration/1 -> State derivative/3
  Pend acceleration/1 -> State derivative/4
  State derivative/1 -> xdot/1

== system furuta_block_model/05 Furuta plant/RK4 Furuta plant/Substep 3/k4 ==
  x : Inport
  tau : Inport  Port=2
  Arm acceleration : Fcn  Expr=(u(3)*u(4)-u(2)*u(5))/(u(1)*u(3)-(u(2)*u(2)))
  Arm rate : Fcn  Expr=u(3)
  D11 : Fcn  Expr=u(6)+u(7)*(sin(u(2))*sin(u(2)))
  D12 : Fcn  Expr=u(9)*cos(u(2))
  D22 : Fcn  Expr=u(8)
  Mass matrix and RHS : Mux  Inputs=5
  Pend acceleration : Fcn  Expr=(u(1)*u(5)-u(2)*u(4))/(u(1)*u(3)-(u(2)*u(2)))
  Pend rate : Fcn  Expr=u(4)
  Physical parameters : Constant  Value=plantCoefficients
  State derivative : Mux
  State torque parameters : Mux  Inputs=3
  Torque RHS arm : Fcn  Expr=u(5)-2*u(7)*sin(u(2))*cos(u(2))*u(3)*u(4)+u(9)*sin(u(2))*(u(4)*u(4))-u(11)*u(3)-u(13)*sgn(u(3))
  Torque RHS pend : Fcn  Expr=u(7)*sin(u(2))*cos(u(2))*(u(3)*u(3))-u(12)*u(4)+u(10)*sin(u(2))
  xdot : Outport
  wires:
  x/1 -> State torque parameters/1
  tau/1 -> State torque parameters/2
  Physical parameters/1 -> State torque parameters/3
  State torque parameters/1 -> D11/1, D12/1, D22/1, Torque RHS arm/1, Torque RHS pend/1, Arm rate/1, Pend rate/1
  D11/1 -> Mass matrix and RHS/1
  D12/1 -> Mass matrix and RHS/2
  D22/1 -> Mass matrix and RHS/3
  Torque RHS arm/1 -> Mass matrix and RHS/4
  Torque RHS pend/1 -> Mass matrix and RHS/5
  Arm rate/1 -> State derivative/1
  Pend rate/1 -> State derivative/2
  Mass matrix and RHS/1 -> Arm acceleration/1, Pend acceleration/1
  Arm acceleration/1 -> State derivative/3
  Pend acceleration/1 -> State derivative/4
  State derivative/1 -> xdot/1

== system furuta_block_model/05 Furuta plant/RK4 Furuta plant/Substep 4/k1 ==
  x : Inport
  tau : Inport  Port=2
  Arm acceleration : Fcn  Expr=(u(3)*u(4)-u(2)*u(5))/(u(1)*u(3)-(u(2)*u(2)))
  Arm rate : Fcn  Expr=u(3)
  D11 : Fcn  Expr=u(6)+u(7)*(sin(u(2))*sin(u(2)))
  D12 : Fcn  Expr=u(9)*cos(u(2))
  D22 : Fcn  Expr=u(8)
  Mass matrix and RHS : Mux  Inputs=5
  Pend acceleration : Fcn  Expr=(u(1)*u(5)-u(2)*u(4))/(u(1)*u(3)-(u(2)*u(2)))
  Pend rate : Fcn  Expr=u(4)
  Physical parameters : Constant  Value=plantCoefficients
  State derivative : Mux
  State torque parameters : Mux  Inputs=3
  Torque RHS arm : Fcn  Expr=u(5)-2*u(7)*sin(u(2))*cos(u(2))*u(3)*u(4)+u(9)*sin(u(2))*(u(4)*u(4))-u(11)*u(3)-u(13)*sgn(u(3))
  Torque RHS pend : Fcn  Expr=u(7)*sin(u(2))*cos(u(2))*(u(3)*u(3))-u(12)*u(4)+u(10)*sin(u(2))
  xdot : Outport
  wires:
  State derivative/1 -> xdot/1
  Pend acceleration/1 -> State derivative/4
  Arm acceleration/1 -> State derivative/3
  Mass matrix and RHS/1 -> Pend acceleration/1, Arm acceleration/1
  Pend rate/1 -> State derivative/2
  Arm rate/1 -> State derivative/1
  Torque RHS pend/1 -> Mass matrix and RHS/5
  Torque RHS arm/1 -> Mass matrix and RHS/4
  D22/1 -> Mass matrix and RHS/3
  D12/1 -> Mass matrix and RHS/2
  D11/1 -> Mass matrix and RHS/1
  State torque parameters/1 -> Pend rate/1, Arm rate/1, Torque RHS pend/1, Torque RHS arm/1, D22/1, D12/1, D11/1
  Physical parameters/1 -> State torque parameters/3
  tau/1 -> State torque parameters/2
  x/1 -> State torque parameters/1

== system furuta_block_model/05 Furuta plant/RK4 Furuta plant/Substep 4/k2 ==
  x : Inport
  tau : Inport  Port=2
  Arm acceleration : Fcn  Expr=(u(3)*u(4)-u(2)*u(5))/(u(1)*u(3)-(u(2)*u(2)))
  Arm rate : Fcn  Expr=u(3)
  D11 : Fcn  Expr=u(6)+u(7)*(sin(u(2))*sin(u(2)))
  D12 : Fcn  Expr=u(9)*cos(u(2))
  D22 : Fcn  Expr=u(8)
  Mass matrix and RHS : Mux  Inputs=5
  Pend acceleration : Fcn  Expr=(u(1)*u(5)-u(2)*u(4))/(u(1)*u(3)-(u(2)*u(2)))
  Pend rate : Fcn  Expr=u(4)
  Physical parameters : Constant  Value=plantCoefficients
  State derivative : Mux
  State torque parameters : Mux  Inputs=3
  Torque RHS arm : Fcn  Expr=u(5)-2*u(7)*sin(u(2))*cos(u(2))*u(3)*u(4)+u(9)*sin(u(2))*(u(4)*u(4))-u(11)*u(3)-u(13)*sgn(u(3))
  Torque RHS pend : Fcn  Expr=u(7)*sin(u(2))*cos(u(2))*(u(3)*u(3))-u(12)*u(4)+u(10)*sin(u(2))
  xdot : Outport
  wires:
  x/1 -> State torque parameters/1
  tau/1 -> State torque parameters/2
  Physical parameters/1 -> State torque parameters/3
  State torque parameters/1 -> D11/1, D12/1, D22/1, Torque RHS arm/1, Torque RHS pend/1, Arm rate/1, Pend rate/1
  D11/1 -> Mass matrix and RHS/1
  D12/1 -> Mass matrix and RHS/2
  D22/1 -> Mass matrix and RHS/3
  Torque RHS arm/1 -> Mass matrix and RHS/4
  Torque RHS pend/1 -> Mass matrix and RHS/5
  Arm rate/1 -> State derivative/1
  Pend rate/1 -> State derivative/2
  Mass matrix and RHS/1 -> Arm acceleration/1, Pend acceleration/1
  Arm acceleration/1 -> State derivative/3
  Pend acceleration/1 -> State derivative/4
  State derivative/1 -> xdot/1

== system furuta_block_model/05 Furuta plant/RK4 Furuta plant/Substep 4/k3 ==
  x : Inport
  tau : Inport  Port=2
  Arm acceleration : Fcn  Expr=(u(3)*u(4)-u(2)*u(5))/(u(1)*u(3)-(u(2)*u(2)))
  Arm rate : Fcn  Expr=u(3)
  D11 : Fcn  Expr=u(6)+u(7)*(sin(u(2))*sin(u(2)))
  D12 : Fcn  Expr=u(9)*cos(u(2))
  D22 : Fcn  Expr=u(8)
  Mass matrix and RHS : Mux  Inputs=5
  Pend acceleration : Fcn  Expr=(u(1)*u(5)-u(2)*u(4))/(u(1)*u(3)-(u(2)*u(2)))
  Pend rate : Fcn  Expr=u(4)
  Physical parameters : Constant  Value=plantCoefficients
  State derivative : Mux
  State torque parameters : Mux  Inputs=3
  Torque RHS arm : Fcn  Expr=u(5)-2*u(7)*sin(u(2))*cos(u(2))*u(3)*u(4)+u(9)*sin(u(2))*(u(4)*u(4))-u(11)*u(3)-u(13)*sgn(u(3))
  Torque RHS pend : Fcn  Expr=u(7)*sin(u(2))*cos(u(2))*(u(3)*u(3))-u(12)*u(4)+u(10)*sin(u(2))
  xdot : Outport
  wires:
  x/1 -> State torque parameters/1
  tau/1 -> State torque parameters/2
  Physical parameters/1 -> State torque parameters/3
  State torque parameters/1 -> D11/1, D12/1, D22/1, Torque RHS arm/1, Torque RHS pend/1, Arm rate/1, Pend rate/1
  D11/1 -> Mass matrix and RHS/1
  D12/1 -> Mass matrix and RHS/2
  D22/1 -> Mass matrix and RHS/3
  Torque RHS arm/1 -> Mass matrix and RHS/4
  Torque RHS pend/1 -> Mass matrix and RHS/5
  Arm rate/1 -> State derivative/1
  Pend rate/1 -> State derivative/2
  Mass matrix and RHS/1 -> Arm acceleration/1, Pend acceleration/1
  Arm acceleration/1 -> State derivative/3
  Pend acceleration/1 -> State derivative/4
  State derivative/1 -> xdot/1

== system furuta_block_model/05 Furuta plant/RK4 Furuta plant/Substep 4/k4 ==
  x : Inport
  tau : Inport  Port=2
  Arm acceleration : Fcn  Expr=(u(3)*u(4)-u(2)*u(5))/(u(1)*u(3)-(u(2)*u(2)))
  Arm rate : Fcn  Expr=u(3)
  D11 : Fcn  Expr=u(6)+u(7)*(sin(u(2))*sin(u(2)))
  D12 : Fcn  Expr=u(9)*cos(u(2))
  D22 : Fcn  Expr=u(8)
  Mass matrix and RHS : Mux  Inputs=5
  Pend acceleration : Fcn  Expr=(u(1)*u(5)-u(2)*u(4))/(u(1)*u(3)-(u(2)*u(2)))
  Pend rate : Fcn  Expr=u(4)
  Physical parameters : Constant  Value=plantCoefficients
  State derivative : Mux
  State torque parameters : Mux  Inputs=3
  Torque RHS arm : Fcn  Expr=u(5)-2*u(7)*sin(u(2))*cos(u(2))*u(3)*u(4)+u(9)*sin(u(2))*(u(4)*u(4))-u(11)*u(3)-u(13)*sgn(u(3))
  Torque RHS pend : Fcn  Expr=u(7)*sin(u(2))*cos(u(2))*(u(3)*u(3))-u(12)*u(4)+u(10)*sin(u(2))
  xdot : Outport
  wires:
  x/1 -> State torque parameters/1
  tau/1 -> State torque parameters/2
  Physical parameters/1 -> State torque parameters/3
  State torque parameters/1 -> D11/1, D12/1, D22/1, Torque RHS arm/1, Torque RHS pend/1, Arm rate/1, Pend rate/1
  D11/1 -> Mass matrix and RHS/1
  D12/1 -> Mass matrix and RHS/2
  D22/1 -> Mass matrix and RHS/3
  Torque RHS arm/1 -> Mass matrix and RHS/4
  Torque RHS pend/1 -> Mass matrix and RHS/5
  Arm rate/1 -> State derivative/1
  Pend rate/1 -> State derivative/2
  Mass matrix and RHS/1 -> Arm acceleration/1, Pend acceleration/1
  Arm acceleration/1 -> State derivative/3
  Pend acceleration/1 -> State derivative/4
  State derivative/1 -> xdot/1

== system furuta_block_model/05 Furuta plant/RK4 Furuta plant/Substep 5/k1 ==
  x : Inport
  tau : Inport  Port=2
  Arm acceleration : Fcn  Expr=(u(3)*u(4)-u(2)*u(5))/(u(1)*u(3)-(u(2)*u(2)))
  Arm rate : Fcn  Expr=u(3)
  D11 : Fcn  Expr=u(6)+u(7)*(sin(u(2))*sin(u(2)))
  D12 : Fcn  Expr=u(9)*cos(u(2))
  D22 : Fcn  Expr=u(8)
  Mass matrix and RHS : Mux  Inputs=5
  Pend acceleration : Fcn  Expr=(u(1)*u(5)-u(2)*u(4))/(u(1)*u(3)-(u(2)*u(2)))
  Pend rate : Fcn  Expr=u(4)
  Physical parameters : Constant  Value=plantCoefficients
  State derivative : Mux
  State torque parameters : Mux  Inputs=3
  Torque RHS arm : Fcn  Expr=u(5)-2*u(7)*sin(u(2))*cos(u(2))*u(3)*u(4)+u(9)*sin(u(2))*(u(4)*u(4))-u(11)*u(3)-u(13)*sgn(u(3))
  Torque RHS pend : Fcn  Expr=u(7)*sin(u(2))*cos(u(2))*(u(3)*u(3))-u(12)*u(4)+u(10)*sin(u(2))
  xdot : Outport
  wires:
  State derivative/1 -> xdot/1
  Pend acceleration/1 -> State derivative/4
  Arm acceleration/1 -> State derivative/3
  Mass matrix and RHS/1 -> Pend acceleration/1, Arm acceleration/1
  Pend rate/1 -> State derivative/2
  Arm rate/1 -> State derivative/1
  Torque RHS pend/1 -> Mass matrix and RHS/5
  Torque RHS arm/1 -> Mass matrix and RHS/4
  D22/1 -> Mass matrix and RHS/3
  D12/1 -> Mass matrix and RHS/2
  D11/1 -> Mass matrix and RHS/1
  State torque parameters/1 -> Pend rate/1, Arm rate/1, Torque RHS pend/1, Torque RHS arm/1, D22/1, D12/1, D11/1
  Physical parameters/1 -> State torque parameters/3
  tau/1 -> State torque parameters/2
  x/1 -> State torque parameters/1

== system furuta_block_model/05 Furuta plant/RK4 Furuta plant/Substep 5/k2 ==
  x : Inport
  tau : Inport  Port=2
  Arm acceleration : Fcn  Expr=(u(3)*u(4)-u(2)*u(5))/(u(1)*u(3)-(u(2)*u(2)))
  Arm rate : Fcn  Expr=u(3)
  D11 : Fcn  Expr=u(6)+u(7)*(sin(u(2))*sin(u(2)))
  D12 : Fcn  Expr=u(9)*cos(u(2))
  D22 : Fcn  Expr=u(8)
  Mass matrix and RHS : Mux  Inputs=5
  Pend acceleration : Fcn  Expr=(u(1)*u(5)-u(2)*u(4))/(u(1)*u(3)-(u(2)*u(2)))
  Pend rate : Fcn  Expr=u(4)
  Physical parameters : Constant  Value=plantCoefficients
  State derivative : Mux
  State torque parameters : Mux  Inputs=3
  Torque RHS arm : Fcn  Expr=u(5)-2*u(7)*sin(u(2))*cos(u(2))*u(3)*u(4)+u(9)*sin(u(2))*(u(4)*u(4))-u(11)*u(3)-u(13)*sgn(u(3))
  Torque RHS pend : Fcn  Expr=u(7)*sin(u(2))*cos(u(2))*(u(3)*u(3))-u(12)*u(4)+u(10)*sin(u(2))
  xdot : Outport
  wires:
  x/1 -> State torque parameters/1
  tau/1 -> State torque parameters/2
  Physical parameters/1 -> State torque parameters/3
  State torque parameters/1 -> D11/1, D12/1, D22/1, Torque RHS arm/1, Torque RHS pend/1, Arm rate/1, Pend rate/1
  D11/1 -> Mass matrix and RHS/1
  D12/1 -> Mass matrix and RHS/2
  D22/1 -> Mass matrix and RHS/3
  Torque RHS arm/1 -> Mass matrix and RHS/4
  Torque RHS pend/1 -> Mass matrix and RHS/5
  Arm rate/1 -> State derivative/1
  Pend rate/1 -> State derivative/2
  Mass matrix and RHS/1 -> Arm acceleration/1, Pend acceleration/1
  Arm acceleration/1 -> State derivative/3
  Pend acceleration/1 -> State derivative/4
  State derivative/1 -> xdot/1

== system furuta_block_model/05 Furuta plant/RK4 Furuta plant/Substep 5/k3 ==
  x : Inport
  tau : Inport  Port=2
  Arm acceleration : Fcn  Expr=(u(3)*u(4)-u(2)*u(5))/(u(1)*u(3)-(u(2)*u(2)))
  Arm rate : Fcn  Expr=u(3)
  D11 : Fcn  Expr=u(6)+u(7)*(sin(u(2))*sin(u(2)))
  D12 : Fcn  Expr=u(9)*cos(u(2))
  D22 : Fcn  Expr=u(8)
  Mass matrix and RHS : Mux  Inputs=5
  Pend acceleration : Fcn  Expr=(u(1)*u(5)-u(2)*u(4))/(u(1)*u(3)-(u(2)*u(2)))
  Pend rate : Fcn  Expr=u(4)
  Physical parameters : Constant  Value=plantCoefficients
  State derivative : Mux
  State torque parameters : Mux  Inputs=3
  Torque RHS arm : Fcn  Expr=u(5)-2*u(7)*sin(u(2))*cos(u(2))*u(3)*u(4)+u(9)*sin(u(2))*(u(4)*u(4))-u(11)*u(3)-u(13)*sgn(u(3))
  Torque RHS pend : Fcn  Expr=u(7)*sin(u(2))*cos(u(2))*(u(3)*u(3))-u(12)*u(4)+u(10)*sin(u(2))
  xdot : Outport
  wires:
  x/1 -> State torque parameters/1
  tau/1 -> State torque parameters/2
  Physical parameters/1 -> State torque parameters/3
  State torque parameters/1 -> D11/1, D12/1, D22/1, Torque RHS arm/1, Torque RHS pend/1, Arm rate/1, Pend rate/1
  D11/1 -> Mass matrix and RHS/1
  D12/1 -> Mass matrix and RHS/2
  D22/1 -> Mass matrix and RHS/3
  Torque RHS arm/1 -> Mass matrix and RHS/4
  Torque RHS pend/1 -> Mass matrix and RHS/5
  Arm rate/1 -> State derivative/1
  Pend rate/1 -> State derivative/2
  Mass matrix and RHS/1 -> Arm acceleration/1, Pend acceleration/1
  Arm acceleration/1 -> State derivative/3
  Pend acceleration/1 -> State derivative/4
  State derivative/1 -> xdot/1

== system furuta_block_model/05 Furuta plant/RK4 Furuta plant/Substep 5/k4 ==
  x : Inport
  tau : Inport  Port=2
  Arm acceleration : Fcn  Expr=(u(3)*u(4)-u(2)*u(5))/(u(1)*u(3)-(u(2)*u(2)))
  Arm rate : Fcn  Expr=u(3)
  D11 : Fcn  Expr=u(6)+u(7)*(sin(u(2))*sin(u(2)))
  D12 : Fcn  Expr=u(9)*cos(u(2))
  D22 : Fcn  Expr=u(8)
  Mass matrix and RHS : Mux  Inputs=5
  Pend acceleration : Fcn  Expr=(u(1)*u(5)-u(2)*u(4))/(u(1)*u(3)-(u(2)*u(2)))
  Pend rate : Fcn  Expr=u(4)
  Physical parameters : Constant  Value=plantCoefficients
  State derivative : Mux
  State torque parameters : Mux  Inputs=3
  Torque RHS arm : Fcn  Expr=u(5)-2*u(7)*sin(u(2))*cos(u(2))*u(3)*u(4)+u(9)*sin(u(2))*(u(4)*u(4))-u(11)*u(3)-u(13)*sgn(u(3))
  Torque RHS pend : Fcn  Expr=u(7)*sin(u(2))*cos(u(2))*(u(3)*u(3))-u(12)*u(4)+u(10)*sin(u(2))
  xdot : Outport
  wires:
  x/1 -> State torque parameters/1
  tau/1 -> State torque parameters/2
  Physical parameters/1 -> State torque parameters/3
  State torque parameters/1 -> D11/1, D12/1, D22/1, Torque RHS arm/1, Torque RHS pend/1, Arm rate/1, Pend rate/1
  D11/1 -> Mass matrix and RHS/1
  D12/1 -> Mass matrix and RHS/2
  D22/1 -> Mass matrix and RHS/3
  Torque RHS arm/1 -> Mass matrix and RHS/4
  Torque RHS pend/1 -> Mass matrix and RHS/5
  Arm rate/1 -> State derivative/1
  Pend rate/1 -> State derivative/2
  Mass matrix and RHS/1 -> Arm acceleration/1, Pend acceleration/1
  Arm acceleration/1 -> State derivative/3
  Pend acceleration/1 -> State derivative/4
  State derivative/1 -> xdot/1

== matlab function furuta_block_model/03 Controllers/PID/PID with anti windup ==
  data: x input; u output; g input; dt input; mode input
function u = pid(x,g,dt,mode)
% 적분은 PID 모드에서만 갱신하고 입력 포화 방향에서는 누적하지 않는다.
persistent integral
if isempty(integral) || mode ~= 2
    integral = 0;
end
e = atan2(sin(x(2)),cos(x(2)));
base = g(1)*e+g(2)*x(4)+g(3)*x(1)+g(4)*x(3);
candidate = base+g(5)*(integral+dt*e);
if mode == 2 && (abs(candidate)<=1 || sign(candidate)~=sign(e))
    integral = integral+dt*e;
end
u = base+g(5)*integral;
end

== matlab function furuta_block_model/03 Controllers/SAC/RL observation reward termination ==
  data: x input; obs output; lastAction input; level input; mode input; reward output; done output
function [obs,reward,done] = observe(x,lastAction,level,mode)
% 상태는 현재 샘플, 보상에 쓰는 행동은 이전 샘플이다.
c = cos(x(2)); s = sin(x(2));
obs = [c;s;x(1);x(3);x(4)];
reward = c-0.01*lastAction^2;
if level == 2
    reward = reward-.001*x(4)^2-.00002*x(3)^2+double(abs(atan2(s,c))<.35);
end
done = mode == 5 && abs(x(1))>2*pi;
if done
    reward = -50;
end
end

== matlab function furuta_block_model/03 Controllers/LMPC (sim)/LMPC bounded QP ==
  data: x input; u output; mode input; H input; F input
function u = move(x,mode,H,F)
% 이전 해를 한 단계 이동해 재사용하고 모든 좌표를 [-1,1]로 제한한다.
persistent previous
if isempty(previous)
    previous = zeros(20,1);
end
u = 0;
if mode ~= 6
    previous(:) = 0;
    return
end
z = x(:);
z(2) = atan2(sin(z(2)),cos(z(2)));
f = F*z;
U = [previous(2:end); previous(end)];
gradient = H*U+f;
for it = 1:100
    change = 0;
    for j = 1:20
        next = min(1,max(-1,U(j)-gradient(j)/H(j,j)));
        step = next-U(j);
        U(j) = next;
        gradient = gradient+H(:,j)*step;
        change = max(change,abs(step));
    end
    if change<1e-7
        break
    end
end
previous = U;
u = U(1);
end

== matlab function furuta_block_model/04 Actuator/RMD X6 P20 60 E/01 RMD Driver/Current PI and duty ==
  data: reference input; duty output; current input; emf input; p input; v output
function [duty,v] = regulate(reference,current,emf,p)
% 3상 등가 q축 전압 제한으로 정규화한 평균 브리지 지령.
persistent integral
if isempty(integral)
    integral = 0;
end
err = reference-current;
raw = emf+p(1)*err+integral;
vmax = p(4)/sqrt(3);
v = max(-vmax,min(vmax,raw));
if abs(raw)<=vmax || sign(raw)~=sign(err)
    integral = integral+p(2)*p(3)*err;
end
duty = .5+.5*v/p(4);
end
